simulink model "robot"  (R2024a)
settings: Solver=VariableStepAuto  StartTime=0.0  StopTime=100  RelTol=1e-3
PreLoadFcn:
  | m = 2.5;
  | k_drag = 30;
  | r = 0.15;
InitFcn:
  | m = 2.5;
  | k_drag = 30;
  | r = 0.15;
StartFcn:
  | m = 2.5;
  | k_drag = 30;
  | r = 0.15;
undefined symbols (not defined in the file): magnitude
libraries: slpidlib x2, simulink x1
settings Model: Creator=Administrator  LastModifiedBy=Administrator

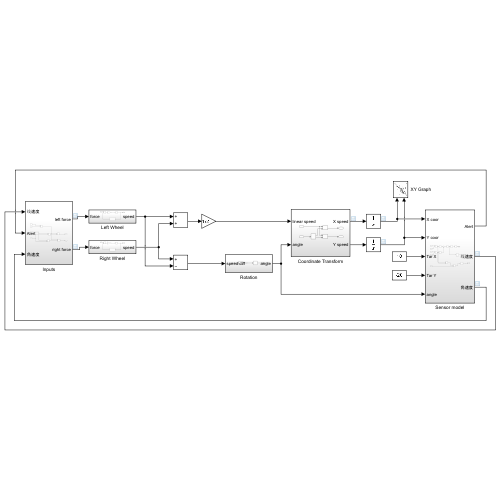
[thumbnail: Simulink's stored preview of the top-level diagram]
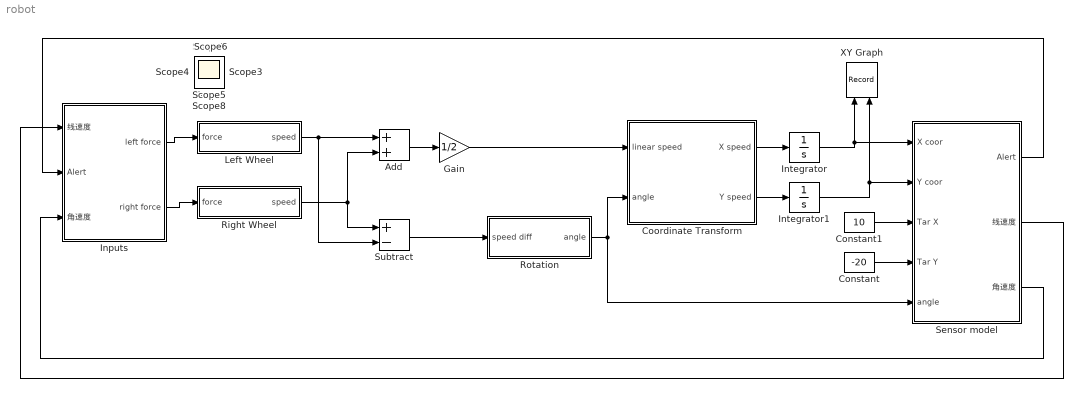
== system robot ==
  Add : Sum
  Constant : Constant  Value=-20
  Constant1 : Constant  Value=10
  Coordinate Transform : Subsystem
  Gain : Gain  Gain=1/2
  Inputs : Subsystem
  Integrator : Integrator
  Integrator1 : Integrator
  Left Wheel : Subsystem
  Right Wheel : Subsystem
  Rotation : Subsystem
  Sensor model : Subsystem
  Subtract : Sum  Inputs=+-
  XY Graph : Record  FileSettingsInternal="{\"entries\":[{\"content\":{\"excelSettings\":{\"content\":{},\"type\":\"Streamout.ExcelSettings\"}},\"type\":\"Streamout.FileSettingStorage\",\"uuid\":\"\"}],\"packageUris\":[\"http:\\/\\/schema.mathworks.com\\/mf0\\/streamout_blocks\\/R2020a\"],\"version\":\"1.0\"}"  Layout=[1 1]  SignalsInternal="{\"entries\":[{\"content\":{\"signals\":[{\"content\":{\"blockPath\":[],\"dimensions\":[1],\"domain\":\"\",\"lineColor\":\"#a2142f\",\"plots\":[ 1 ],\"port\":1,\"sid\":[\"\"],\"signalID\":1,\"signalName\":\"Integrator\"},\"type\":\"RecordBlkView.Signal\",\"uuid\":\"\"},{\"content\":{\"blockPath\":[],\"dimensions\":[1],\"domain\":\"\",\"lineColor\":\"#139fff\",\"plots\":[ 1 ],\"port\":2,\"sid\":[\"\"],\"signalID\":2,\"signalName\":\"Integrator1\"},\"type\":\"RecordBlkView.Signal\",\"uuid\":\"\"}]},\"type\":\"RecordBlkView.InputSignals\",\"uuid\":\"\"}],\"packageUris\":[\"http:\\/\\/schema.mathworks.com\\/mf0\\/streamout_blocks\\/R2020a\"],\"version\":\"1.0\"}"  VisualizationBindings="{\"xyplotplugin\":{\"info\":[{\"series\":[{\"bindingParametersList\":[{\"parameter\":\"X-Axis\",\"signalID\":1,\"signalName\":\"Integrator\"},{\"parameter\":\"Y-Axis\",\"signalID\":2,\"signalName\":\"Integrator1\"}],\"seriesID\":0}],\"subplotID\":1}]}}"  CompatibilityTag=XY
  Scope{,1..6,8} (8 alike) : Scope
  wires:
  Right Wheel/1(speed) -> Subtract/1, Add/2
  Add/1 -> Gain/1
  Coordinate Transform/1(X speed) -> Integrator/1
  Coordinate Transform/2(Y speed) -> Integrator1/1
  Inputs/2(right force) -> Right Wheel/1(force)
  Subtract/1 -> Rotation/1(speed diff)
  Gain/1 -> Coordinate Transform/1(linear speed)
  Rotation/1(angle) -> Coordinate Transform/2(angle), Sensor model/5(angle)
  Inputs/1(left force) -> Left Wheel/1(force)
  Left Wheel/1(speed) -> Subtract/2, Add/1
  Integrator1/1 -> Sensor model/2(Y coor), XY Graph/2
  Integrator/1 -> Sensor model/1(X coor), XY Graph/1
  Constant/1 -> Sensor model/4(Tar Y)
  Constant1/1 -> Sensor model/3(Tar X)
  Sensor model/2(线速度) -> Inputs/1(线速度)
  Sensor model/3(角速度) -> Inputs/3(角速度)
  Sensor model/1(Alert) -> Inputs/2(Alert)

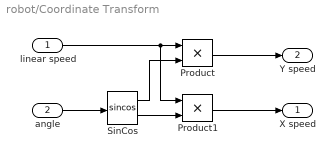
== system robot/Coordinate Transform ==
  linear speed : Inport
  angle : Inport  Port=2
  Product : Product
  Product1 : Product
  SinCos : Trigonometry  Operator=sincos
  X speed : Outport
  Y speed : Outport  Port=2
  wires:
  angle/1 -> SinCos/1
  linear speed/1 -> Product1/1, Product/1
  SinCos/1 -> Product/2
  SinCos/2 -> Product1/2
  Product/1 -> Y speed/1
  Product1/1 -> X speed/1

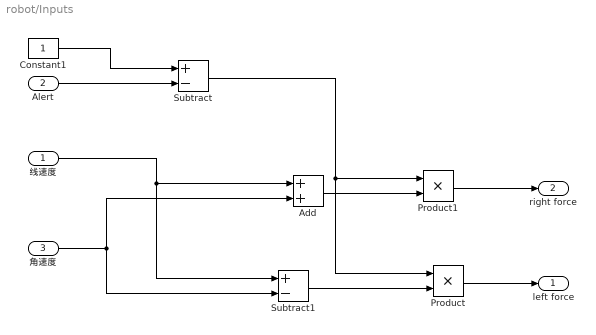
== system robot/Inputs ==
  线速度 : Inport
  Alert : Inport  Port=2
  角速度 : Inport  Port=3
  Add : Sum
  Constant1 : Constant
  Product : Product
  Product1 : Product
  Subtract : Sum  Inputs=+-
  Subtract1 : Sum  Inputs=+-
  left force : Outport
  right force : Outport  Port=2
  wires:
  Constant1/1 -> Subtract/1
  Alert/1 -> Subtract/2
  Subtract/1 -> Product1/1, Product/1
  Add/1 -> Product1/2
  Subtract1/1 -> Product/2
  线速度/1 -> Add/1, Subtract1/1
  角速度/1 -> Add/2, Subtract1/2
  Product1/1 -> right force/1
  Product/1 -> left force/1

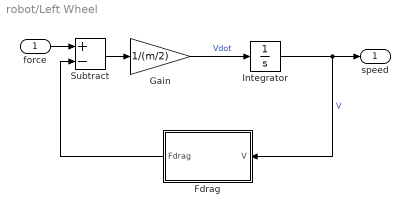
== system robot/Left Wheel ==
  force : Inport
  Fdrag : MATLAB Function  TreatAsAtomicUnit=on
  Gain : Gain  Gain=1/(m/2)
  Integrator : Integrator
  Subtract : Sum  Inputs=+-
  speed : Outport
  wires:
  Subtract/1 -> Gain/1
  Integrator/1 -> speed/1, Fdrag/1(V)  "V"
  Fdrag/1(Fdrag) -> Subtract/2
  force/1 -> Subtract/1
  Gain/1 -> Integrator/1  "Vdot"

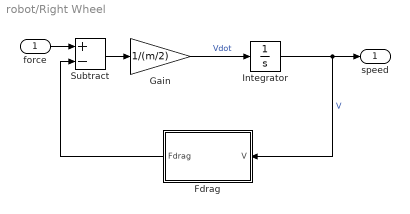
== system robot/Right Wheel ==
  force : Inport
  Fdrag : MATLAB Function  TreatAsAtomicUnit=on
  Gain : Gain  Gain=1/(m/2)
  Integrator : Integrator
  Subtract : Sum  Inputs=+-
  speed : Outport
  wires:
  Gain/1 -> Integrator/1  "Vdot"
  Integrator/1 -> speed/1, Fdrag/1(V)  "V"
  force/1 -> Subtract/1
  Subtract/1 -> Gain/1
  Fdrag/1(Fdrag) -> Subtract/2

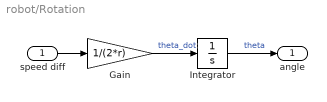
== system robot/Rotation ==
  speed diff : Inport
  Gain : Gain  Gain=1/(2*r)
  Integrator : Integrator
  angle : Outport
  wires:
  speed diff/1 -> Gain/1
  Gain/1 -> Integrator/1  "theta_dot"
  Integrator/1 -> angle/1  "theta"

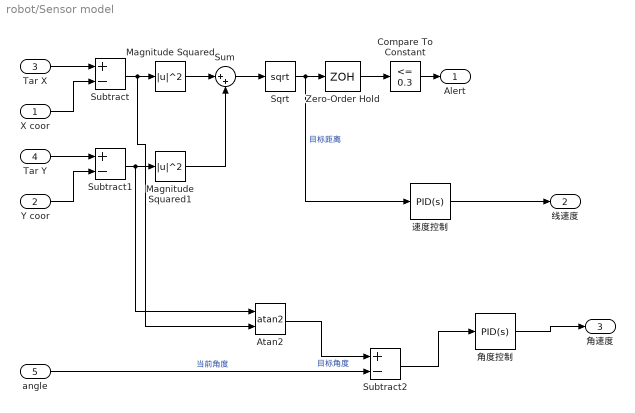
== system robot/Sensor model ==
  X coor : Inport
  Y coor : Inport  Port=2
  Tar X : Inport  Port=3
  Tar Y : Inport  Port=4
  angle : Inport  Port=5
  Atan2 : Trigonometry  Operator=atan2
  Compare To Constant : simulink/Logic and Bit Operations/Compare To Constant  relop=<=  const=0.3  OutDataTypeStr=boolean
  Magnitude Squared : Math  Operator=magnitude^2
  Magnitude Squared1 : Math  Operator=magnitude^2
  Sqrt : Sqrt
  Subtract : Sum  Inputs=+-
  Subtract1 : Sum  Inputs=+-
  Subtract2 : Sum  Inputs=+-
  Sum : Sum  Inputs=|++
  Zero-Order Hold : ZeroOrderHold  SampleTime=0.25
  角度控制 : slpidlib/PID Controller  Controller=PID  Form=Parallel  TimeDomain=Continuous-time  UseExternalTs=off  SampleTime=-1  IntegratorMethod=Forward Euler  FilterMethod=Forward Euler  ControllerParametersSource=internal  P=10  I=0  UseKiTs=off  D=1  UseExternalDerivativeSource=off  N=100  UseFilter=on  TunerSelectOption=Transfer Function Based (PID Tuner App)  InitialConditionSource=internal  InitialConditionForIntegrator=0  InitialConditionForFilter=0  DifferentiatorICPrevScaledInput=0  ExternalReset=none  TrackingMode=off  Kt=1  LimitOutput=on  SatLimitsSource=internal  UpperSaturationLimit=2  LowerSaturationLimit=-2  LinearizeAsGain=on  AntiWindupMode=none  Kb=1  LimitIntegrator=off  UpperIntegratorSaturationLimit=inf  LowerIntegratorSaturationLimit=-inf  POutMin=[]  POutMax=[]  IOutMin=[]  IOutMax=[]  DOutMin=[]  DOutMax=[]  NOutMin=[]  NOutMax=[]  SumOutMin=[]  SumOutMax=[]  SaturationOutMin=[]  SaturationOutMax=[]  PParamMin=[]  PParamMax=[]  IParamMin=[]  IParamMax=[]  DParamMin=[]  DParamMax=[]  NParamMin=[]  NParamMax=[]  KbParamMin=[]  KbParamMax=[]  KtParamMin=[]  KtParamMax=[]  KbOutMin=[]  KbOutMax=[]  KtOutMin=[]  KtOutMax=[]  IntegratorOutMin=[]  IntegratorOutMax=[]  FilterOutMin=[]  FilterOutMax=[]  SumI1OutMin=[]  SumI1OutMax=[]  SumI2OutMin=[]  SumI2OutMax=[]  SumI3OutMin=[]  SumI3OutMax=[]  SumI4OutMin=[]  SumI4OutMax=[]  SumDOutMin=[]  SumDOutMax=[]  DifferentiatorOutMin=[]  DifferentiatorOutMax=[]  FilterDiffOutCoefMin=[]  FilterDiffOutCoefMax=[]  ReciprocalOutMin=[]  ReciprocalOutMax=[]  SumDenOutMin=[]  SumDenOutMax=[]  SumNumOutMin=[]  SumNumOutMax=[]  DivideOutMin=[]  DivideOutMax=[]  UdiffTsProdOutMin=[]  UdiffTsProdOutMax=[]  NTsProdOutMin=[]  NTsProdOutMax=[]  UintegralTsProdOutMin=[]  UintegralTsProdOutMax=[]  UngainTsProdOutMin=[]  UngainTsProdOutMax=[]  ClampingZeroOutDataTypeStr=Inherit: Inherit via back propagation  ClampingZeroOutMin=[]  ClampingZeroOutMax=[]  FilterDenConstantOutDataTypeStr=Inherit: Inherit via back propagation  FilterDenConstantOutMin=[]  FilterDenConstantOutMax=[]  PCopyOutDataTypeStr=Inherit: Inherit via back propagation  PCopyOutMin=[]  PCopyOutMax=[]  NCopyOutDataTypeStr=Inherit: Inherit via back propagation  NCopyOutMin=[]  NCopyOutMax=[]  IntegratorContinuousStateAttributes=''  IntegratorStateMustResolveToSignalObject=off  IntegratorRTWStateStorageClass=Auto  FilterContinuousStateAttributes=''  FilterStateMustResolveToSignalObject=off  FilterRTWStateStorageClass=Auto  ParallelPVariant=InternalParameters  IdealPVariant=Disabled  IVariant=InternalParameters  DVariant=InternalParameters  IntegratorVariant=Continuous  SatVariant=Enabled  AWVariant=Passthrough  PCopyVariant=Disabled  TRVariant=Disabled  FdbkBlocksVariant=Forward  IdealPFdbkVariant=Disabled  SatFdbkVariant=Disabled  DerivativeFilterVariant=ContFilter  NVariant=InternalParameters  NCopyVariant=Disabled  FilterICVariant=InternalICsFilter  IntegratorICVariant=InternalICs  ExternalResetVariant=Disabled  TRSumVariant=Passthrough  SumFdbkVariant=Disabled  SumVariant=Sum_PID  TsampFilterVariant=InternalTs  TsampNgainVariant=Passthrough  TsampIntegralVariant=Disabled_SignalSpec  ExternalSaturationOutDataTypeStr=Inherit: Same as second input  DerivativeSourceVariant=ErrorSignal
  速度控制 : slpidlib/PID Controller  Controller=PID  Form=Parallel  TimeDomain=Continuous-time  UseExternalTs=off  SampleTime=-1  IntegratorMethod=Forward Euler  FilterMethod=Forward Euler  ControllerParametersSource=internal  P=10  I=0  UseKiTs=off  D=1  UseExternalDerivativeSource=off  N=1000  UseFilter=on  TunerSelectOption=Transfer Function Based (PID Tuner App)  InitialConditionSource=internal  InitialConditionForIntegrator=0  InitialConditionForFilter=0  DifferentiatorICPrevScaledInput=0  ExternalReset=none  TrackingMode=off  Kt=1  LimitOutput=on  SatLimitsSource=internal  UpperSaturationLimit=10  LowerSaturationLimit=-10  LinearizeAsGain=on  AntiWindupMode=none  Kb=1  LimitIntegrator=off  UpperIntegratorSaturationLimit=inf  LowerIntegratorSaturationLimit=-inf  POutMin=[]  POutMax=[]  IOutMin=[]  IOutMax=[]  DOutMin=[]  DOutMax=[]  NOutMin=[]  NOutMax=[]  SumOutMin=[]  SumOutMax=[]  SaturationOutMin=[]  SaturationOutMax=[]  PParamMin=[]  PParamMax=[]  IParamMin=[]  IParamMax=[]  DParamMin=[]  DParamMax=[]  NParamMin=[]  NParamMax=[]  KbParamMin=[]  KbParamMax=[]  KtParamMin=[]  KtParamMax=[]  KbOutMin=[]  KbOutMax=[]  KtOutMin=[]  KtOutMax=[]  IntegratorOutMin=[]  IntegratorOutMax=[]  FilterOutMin=[]  FilterOutMax=[]  SumI1OutMin=[]  SumI1OutMax=[]  SumI2OutMin=[]  SumI2OutMax=[]  SumI3OutMin=[]  SumI3OutMax=[]  SumI4OutMin=[]  SumI4OutMax=[]  SumDOutMin=[]  SumDOutMax=[]  DifferentiatorOutMin=[]  DifferentiatorOutMax=[]  FilterDiffOutCoefMin=[]  FilterDiffOutCoefMax=[]  ReciprocalOutMin=[]  ReciprocalOutMax=[]  SumDenOutMin=[]  SumDenOutMax=[]  SumNumOutMin=[]  SumNumOutMax=[]  DivideOutMin=[]  DivideOutMax=[]  UdiffTsProdOutMin=[]  UdiffTsProdOutMax=[]  NTsProdOutMin=[]  NTsProdOutMax=[]  UintegralTsProdOutMin=[]  UintegralTsProdOutMax=[]  UngainTsProdOutMin=[]  UngainTsProdOutMax=[]  ClampingZeroOutDataTypeStr=Inherit: Inherit via back propagation  ClampingZeroOutMin=[]  ClampingZeroOutMax=[]  FilterDenConstantOutDataTypeStr=Inherit: Inherit via back propagation  FilterDenConstantOutMin=[]  FilterDenConstantOutMax=[]  PCopyOutDataTypeStr=Inherit: Inherit via back propagation  PCopyOutMin=[]  PCopyOutMax=[]  NCopyOutDataTypeStr=Inherit: Inherit via back propagation  NCopyOutMin=[]  NCopyOutMax=[]  IntegratorContinuousStateAttributes=''  IntegratorStateMustResolveToSignalObject=off  IntegratorRTWStateStorageClass=Auto  FilterContinuousStateAttributes=''  FilterStateMustResolveToSignalObject=off  FilterRTWStateStorageClass=Auto  ParallelPVariant=InternalParameters  IdealPVariant=Disabled  IVariant=InternalParameters  DVariant=InternalParameters  IntegratorVariant=Continuous  SatVariant=Enabled  AWVariant=Passthrough  PCopyVariant=Disabled  TRVariant=Disabled  FdbkBlocksVariant=Forward  IdealPFdbkVariant=Disabled  SatFdbkVariant=Disabled  DerivativeFilterVariant=ContFilter  NVariant=InternalParameters  NCopyVariant=Disabled  FilterICVariant=InternalICsFilter  IntegratorICVariant=InternalICs  ExternalResetVariant=Disabled  TRSumVariant=Passthrough  SumFdbkVariant=Disabled  SumVariant=Sum_PID  TsampFilterVariant=InternalTs  TsampNgainVariant=Passthrough  TsampIntegralVariant=Disabled_SignalSpec  ExternalSaturationOutDataTypeStr=Inherit: Same as second input  DerivativeSourceVariant=ErrorSignal
  Alert : Outport
  线速度 : Outport  Port=2
  角速度 : Outport  Port=3
  wires:
  X coor/1 -> Subtract/2
  Tar X/1 -> Subtract/1
  Y coor/1 -> Subtract1/2
  Tar Y/1 -> Subtract1/1
  Subtract/1 -> Atan2/2, Magnitude Squared/1
  Magnitude Squared/1 -> Sum/1
  Magnitude Squared1/1 -> Sum/2
  Sum/1 -> Sqrt/1
  Sqrt/1 -> 速度控制/1, Zero-Order Hold/1  "目标距离"
  Zero-Order Hold/1 -> Compare To Constant/1
  Compare To Constant/1 -> Alert/1
  Subtract1/1 -> Atan2/1, Magnitude Squared1/1
  Atan2/1 -> Subtract2/1  "目标角度"
  angle/1 -> Subtract2/2  "当前角度"
  Subtract2/1 -> 角度控制/1
  速度控制/1 -> 线速度/1
  角度控制/1 -> 角速度/1

== matlab function robot/Right Wheel/Fdrag ==
  data: V input; Fdrag output; k_drag parameter
function Fdrag = get_fdrag(V,k_drag)
Fdrag=k_drag*V*abs(V);
end

== matlab function robot/Left Wheel/Fdrag ==
  data: V input; Fdrag output; k_drag parameter
function Fdrag = get_fdrag(V,k_drag)
Fdrag=k_drag*V*abs(V);
end
